simulink model "RobotDelta"  (R2025b)
settings: Solver=VariableStepAuto  StartTime=0.0  StopTime=10.0  RelTol=1e-3
model workspace: external: MATLAB File RobotDelta_DataFile.m (data not in the file)
undefined symbols (not defined in the file or in its folder): smiData, X, Y, Z
libraries: sm_lib x265, nesl_utility x1
(part 4 of 5)

== system RobotDelta/Mat_Bich_8mm_8_RIGID ==
  ReferenceFrame : sm_lib/Frames and Transforms/Reference Frame
  Solid : sm_lib/Body Elements/File Solid  ExtGeomFileName=Mat_Bich_8mm_Default_sldprt.STEP  UnitType=FromFile  ExtGeomFileUnits=m  StepReaderType=HEX  ExportConvexHullGeometry=off  InertiaType=Custom  BasedOnType=DensityFromFile  Density=1000  DensityUnits=kg/m^3  Mass=smiData.Solid(12).mass  MassUnits=kg  CenterOfMass=smiData.Solid(12).CoM  CenterOfMassUnits=mm  MomentsOfInertia=smiData.Solid(12).MoI  MomentsOfInertiaUnits=kg*mm^2  ProductsOfInertia=smiData.Solid(12).PoI  ProductsOfInertiaUnits=kg*mm^2  GraphicType=FromGeometry  MarkerShape=Sphere  MarkerSize=10  GraphicVisPropType=SimpleVisualProperties  GraphicDiffuseColor=smiData.Solid(12).color  GraphicOpacity=smiData.Solid(12).opacity  GraphicSpecularColor=[0.5 0.5 0.5 1.0]  GraphicAmbientColor=[0.15 0.15 0.15 1.0]  GraphicEmissiveColor=[0.0 0.0 0.0 1.0]  GraphicShininess=75  DoExposeReferenceFrame=on  SerializedFrames=<Frames/>
  Transform : sm_lib/Frames and Transforms/Rigid Transform  RotationMethod=ArbitraryAxis  FollAlignAxisA=+X  BaseAlignAxisA=+Y  FollAlignAxisB=+Y  BaseAlignAxisB=+Z  RotationStandardAxis=+Z  RotationAngle=smiData.RigidTransform(56).angle  RotationAngleUnits=rad  RotationArbitraryAxis=smiData.RigidTransform(56).axis  RotationSequenceAxes=FollowerAxes  RotationSequence=XYX  RotationSequenceAngles=[0 0 0]  RotationSequenceAnglesUnits=deg  RotationMatrix=[1 0 0;0 1 0;0 0 1]  Quaternion=[1 0 0 0]  TranslationMethod=Cartesian  TranslationCartesianOffset=smiData.RigidTransform(56).translation  TranslationCartesianOffsetUnits=mm  TranslationStandardAxis=+Z  TranslationStandardOffset=0  TranslationStandardOffsetUnits=m  TranslationROffset=0  TranslationROffsetUnits=m  TranslationThetaOffset=0  TranslationThetaOffsetUnits=deg  TranslationZOffset=0  TranslationZOffsetUnits=m
  Transform1 : sm_lib/Frames and Transforms/Rigid Transform  RotationMethod=ArbitraryAxis  FollAlignAxisA=+X  BaseAlignAxisA=+Y  FollAlignAxisB=+Y  BaseAlignAxisB=+Z  RotationStandardAxis=+Z  RotationAngle=smiData.RigidTransform(58).angle  RotationAngleUnits=rad  RotationArbitraryAxis=smiData.RigidTransform(58).axis  RotationSequenceAxes=FollowerAxes  RotationSequence=XYX  RotationSequenceAngles=[0 0 0]  RotationSequenceAnglesUnits=deg  RotationMatrix=[1 0 0;0 1 0;0 0 1]  Quaternion=[1 0 0 0]  TranslationMethod=Cartesian  TranslationCartesianOffset=smiData.RigidTransform(58).translation  TranslationCartesianOffsetUnits=mm  TranslationStandardAxis=+Z  TranslationStandardOffset=0  TranslationStandardOffsetUnits=m  TranslationROffset=0  TranslationROffsetUnits=m  TranslationThetaOffset=0  TranslationThetaOffsetUnits=deg  TranslationZOffset=0  TranslationZOffsetUnits=m
  F : PMIOPort  Side=Left
  F1 : PMIOPort  Port=2  Side=Left
  connections:
  Solid/RConn1 -- ReferenceFrame/RConn1 -- Transform/LConn1 -- Transform1/LConn1
  Transform/RConn1 -- F/RConn1
  Transform1/RConn1 -- F1/RConn1

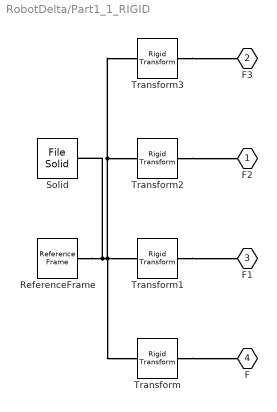
== system RobotDelta/Part1_1_RIGID ==
  ReferenceFrame : sm_lib/Frames and Transforms/Reference Frame
  Solid : sm_lib/Body Elements/File Solid  ExtGeomFileName=Part1_Default_sldprt.STEP  UnitType=FromFile  ExtGeomFileUnits=m  StepReaderType=HEX  ExportConvexHullGeometry=off  InertiaType=Custom  BasedOnType=DensityFromFile  Density=1000  DensityUnits=kg/m^3  Mass=smiData.Solid(10).mass  MassUnits=kg  CenterOfMass=smiData.Solid(10).CoM  CenterOfMassUnits=mm  MomentsOfInertia=smiData.Solid(10).MoI  MomentsOfInertiaUnits=kg*mm^2  ProductsOfInertia=smiData.Solid(10).PoI  ProductsOfInertiaUnits=kg*mm^2  GraphicType=FromGeometry  MarkerShape=Sphere  MarkerSize=10  GraphicVisPropType=SimpleVisualProperties  GraphicDiffuseColor=smiData.Solid(10).color  GraphicOpacity=smiData.Solid(10).opacity  GraphicSpecularColor=[0.5 0.5 0.5 1.0]  GraphicAmbientColor=[0.15 0.15 0.15 1.0]  GraphicEmissiveColor=[0.0 0.0 0.0 1.0]  GraphicShininess=75  DoExposeReferenceFrame=on  SerializedFrames=<Frames/>
  Transform : sm_lib/Frames and Transforms/Rigid Transform  RotationMethod=ArbitraryAxis  FollAlignAxisA=+X  BaseAlignAxisA=+Y  FollAlignAxisB=+Y  BaseAlignAxisB=+Z  RotationStandardAxis=+Z  RotationAngle=smiData.RigidTransform(43).angle  RotationAngleUnits=rad  RotationArbitraryAxis=smiData.RigidTransform(43).axis  RotationSequenceAxes=FollowerAxes  RotationSequence=XYX  RotationSequenceAngles=[0 0 0]  RotationSequenceAnglesUnits=deg  RotationMatrix=[1 0 0;0 1 0;0 0 1]  Quaternion=[1 0 0 0]  TranslationMethod=Cartesian  TranslationCartesianOffset=smiData.RigidTransform(43).translation  TranslationCartesianOffsetUnits=mm  TranslationStandardAxis=+Z  TranslationStandardOffset=0  TranslationStandardOffsetUnits=m  TranslationROffset=0  TranslationROffsetUnits=m  TranslationThetaOffset=0  TranslationThetaOffsetUnits=deg  TranslationZOffset=0  TranslationZOffsetUnits=m
  Transform1 : sm_lib/Frames and Transforms/Rigid Transform  RotationMethod=ArbitraryAxis  FollAlignAxisA=+X  BaseAlignAxisA=+Y  FollAlignAxisB=+Y  BaseAlignAxisB=+Z  RotationStandardAxis=+Z  RotationAngle=smiData.RigidTransform(49).angle  RotationAngleUnits=rad  RotationArbitraryAxis=smiData.RigidTransform(49).axis  RotationSequenceAxes=FollowerAxes  RotationSequence=XYX  RotationSequenceAngles=[0 0 0]  RotationSequenceAnglesUnits=deg  RotationMatrix=[1 0 0;0 1 0;0 0 1]  Quaternion=[1 0 0 0]  TranslationMethod=Cartesian  TranslationCartesianOffset=smiData.RigidTransform(49).translation  TranslationCartesianOffsetUnits=mm  TranslationStandardAxis=+Z  TranslationStandardOffset=0  TranslationStandardOffsetUnits=m  TranslationROffset=0  TranslationROffsetUnits=m  TranslationThetaOffset=0  TranslationThetaOffsetUnits=deg  TranslationZOffset=0  TranslationZOffsetUnits=m
  Transform2 : sm_lib/Frames and Transforms/Rigid Transform  RotationMethod=ArbitraryAxis  FollAlignAxisA=+X  BaseAlignAxisA=+Y  FollAlignAxisB=+Y  BaseAlignAxisB=+Z  RotationStandardAxis=+Z  RotationAngle=smiData.RigidTransform(91).angle  RotationAngleUnits=rad  RotationArbitraryAxis=smiData.RigidTransform(91).axis  RotationSequenceAxes=FollowerAxes  RotationSequence=XYX  RotationSequenceAngles=[0 0 0]  RotationSequenceAnglesUnits=deg  RotationMatrix=[1 0 0;0 1 0;0 0 1]  Quaternion=[1 0 0 0]  TranslationMethod=Cartesian  TranslationCartesianOffset=smiData.RigidTransform(91).translation  TranslationCartesianOffsetUnits=mm  TranslationStandardAxis=+Z  TranslationStandardOffset=0  TranslationStandardOffsetUnits=m  TranslationROffset=0  TranslationROffsetUnits=m  TranslationThetaOffset=0  TranslationThetaOffsetUnits=deg  TranslationZOffset=0  TranslationZOffsetUnits=m
  Transform3 : sm_lib/Frames and Transforms/Rigid Transform  RotationMethod=ArbitraryAxis  FollAlignAxisA=+X  BaseAlignAxisA=+Y  FollAlignAxisB=+Y  BaseAlignAxisB=+Z  RotationStandardAxis=+Z  RotationAngle=smiData.RigidTransform(94).angle  RotationAngleUnits=rad  RotationArbitraryAxis=smiData.RigidTransform(94).axis  RotationSequenceAxes=FollowerAxes  RotationSequence=XYX  RotationSequenceAngles=[0 0 0]  RotationSequenceAnglesUnits=deg  RotationMatrix=[1 0 0;0 1 0;0 0 1]  Quaternion=[1 0 0 0]  TranslationMethod=Cartesian  TranslationCartesianOffset=smiData.RigidTransform(94).translation  TranslationCartesianOffsetUnits=mm  TranslationStandardAxis=+Z  TranslationStandardOffset=0  TranslationStandardOffsetUnits=m  TranslationROffset=0  TranslationROffsetUnits=m  TranslationThetaOffset=0  TranslationThetaOffsetUnits=deg  TranslationZOffset=0  TranslationZOffsetUnits=m
  F2 : PMIOPort  Side=Left
  F3 : PMIOPort  Port=2  Side=Left
  F1 : PMIOPort  Port=3  Side=Left
  F : PMIOPort  Port=4  Side=Left
  connections:
  Solid/RConn1 -- ReferenceFrame/RConn1 -- Transform2/LConn1 -- Transform3/LConn1 -- Transform/LConn1 -- Transform1/LConn1
  Transform/RConn1 -- F/RConn1
  Transform1/RConn1 -- F1/RConn1
  Transform2/RConn1 -- F2/RConn1
  Transform3/RConn1 -- F3/RConn1

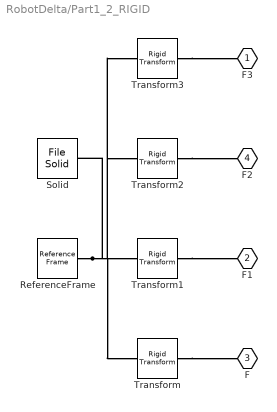
== system RobotDelta/Part1_2_RIGID ==
  ReferenceFrame : sm_lib/Frames and Transforms/Reference Frame
  Solid : sm_lib/Body Elements/File Solid  ExtGeomFileName=Part1_Default_sldprt.STEP  UnitType=FromFile  ExtGeomFileUnits=m  StepReaderType=HEX  ExportConvexHullGeometry=off  InertiaType=Custom  BasedOnType=DensityFromFile  Density=1000  DensityUnits=kg/m^3  Mass=smiData.Solid(10).mass  MassUnits=kg  CenterOfMass=smiData.Solid(10).CoM  CenterOfMassUnits=mm  MomentsOfInertia=smiData.Solid(10).MoI  MomentsOfInertiaUnits=kg*mm^2  ProductsOfInertia=smiData.Solid(10).PoI  ProductsOfInertiaUnits=kg*mm^2  GraphicType=FromGeometry  MarkerShape=Sphere  MarkerSize=10  GraphicVisPropType=SimpleVisualProperties  GraphicDiffuseColor=smiData.Solid(10).color  GraphicOpacity=smiData.Solid(10).opacity  GraphicSpecularColor=[0.5 0.5 0.5 1.0]  GraphicAmbientColor=[0.15 0.15 0.15 1.0]  GraphicEmissiveColor=[0.0 0.0 0.0 1.0]  GraphicShininess=75  DoExposeReferenceFrame=on  SerializedFrames=<Frames/>
  Transform : sm_lib/Frames and Transforms/Rigid Transform  RotationMethod=ArbitraryAxis  FollAlignAxisA=+X  BaseAlignAxisA=+Y  FollAlignAxisB=+Y  BaseAlignAxisB=+Z  RotationStandardAxis=+Z  RotationAngle=smiData.RigidTransform(51).angle  RotationAngleUnits=rad  RotationArbitraryAxis=smiData.RigidTransform(51).axis  RotationSequenceAxes=FollowerAxes  RotationSequence=XYX  RotationSequenceAngles=[0 0 0]  RotationSequenceAnglesUnits=deg  RotationMatrix=[1 0 0;0 1 0;0 0 1]  Quaternion=[1 0 0 0]  TranslationMethod=Cartesian  TranslationCartesianOffset=smiData.RigidTransform(51).translation  TranslationCartesianOffsetUnits=mm  TranslationStandardAxis=+Z  TranslationStandardOffset=0  TranslationStandardOffsetUnits=m  TranslationROffset=0  TranslationROffsetUnits=m  TranslationThetaOffset=0  TranslationThetaOffsetUnits=deg  TranslationZOffset=0  TranslationZOffsetUnits=m
  Transform1 : sm_lib/Frames and Transforms/Rigid Transform  RotationMethod=ArbitraryAxis  FollAlignAxisA=+X  BaseAlignAxisA=+Y  FollAlignAxisB=+Y  BaseAlignAxisB=+Z  RotationStandardAxis=+Z  RotationAngle=smiData.RigidTransform(55).angle  RotationAngleUnits=rad  RotationArbitraryAxis=smiData.RigidTransform(55).axis  RotationSequenceAxes=FollowerAxes  RotationSequence=XYX  RotationSequenceAngles=[0 0 0]  RotationSequenceAnglesUnits=deg  RotationMatrix=[1 0 0;0 1 0;0 0 1]  Quaternion=[1 0 0 0]  TranslationMethod=Cartesian  TranslationCartesianOffset=smiData.RigidTransform(55).translation  TranslationCartesianOffsetUnits=mm  TranslationStandardAxis=+Z  TranslationStandardOffset=0  TranslationStandardOffsetUnits=m  TranslationROffset=0  TranslationROffsetUnits=m  TranslationThetaOffset=0  TranslationThetaOffsetUnits=deg  TranslationZOffset=0  TranslationZOffsetUnits=m
  Transform2 : sm_lib/Frames and Transforms/Rigid Transform  RotationMethod=ArbitraryAxis  FollAlignAxisA=+X  BaseAlignAxisA=+Y  FollAlignAxisB=+Y  BaseAlignAxisB=+Z  RotationStandardAxis=+Z  RotationAngle=smiData.RigidTransform(95).angle  RotationAngleUnits=rad  RotationArbitraryAxis=smiData.RigidTransform(95).axis  RotationSequenceAxes=FollowerAxes  RotationSequence=XYX  RotationSequenceAngles=[0 0 0]  RotationSequenceAnglesUnits=deg  RotationMatrix=[1 0 0;0 1 0;0 0 1]  Quaternion=[1 0 0 0]  TranslationMethod=Cartesian  TranslationCartesianOffset=smiData.RigidTransform(95).translation  TranslationCartesianOffsetUnits=mm  TranslationStandardAxis=+Z  TranslationStandardOffset=0  TranslationStandardOffsetUnits=m  TranslationROffset=0  TranslationROffsetUnits=m  TranslationThetaOffset=0  TranslationThetaOffsetUnits=deg  TranslationZOffset=0  TranslationZOffsetUnits=m
  Transform3 : sm_lib/Frames and Transforms/Rigid Transform  RotationMethod=ArbitraryAxis  FollAlignAxisA=+X  BaseAlignAxisA=+Y  FollAlignAxisB=+Y  BaseAlignAxisB=+Z  RotationStandardAxis=+Z  RotationAngle=smiData.RigidTransform(98).angle  RotationAngleUnits=rad  RotationArbitraryAxis=smiData.RigidTransform(98).axis  RotationSequenceAxes=FollowerAxes  RotationSequence=XYX  RotationSequenceAngles=[0 0 0]  RotationSequenceAnglesUnits=deg  RotationMatrix=[1 0 0;0 1 0;0 0 1]  Quaternion=[1 0 0 0]  TranslationMethod=Cartesian  TranslationCartesianOffset=smiData.RigidTransform(98).translation  TranslationCartesianOffsetUnits=mm  TranslationStandardAxis=+Z  TranslationStandardOffset=0  TranslationStandardOffsetUnits=m  TranslationROffset=0  TranslationROffsetUnits=m  TranslationThetaOffset=0  TranslationThetaOffsetUnits=deg  TranslationZOffset=0  TranslationZOffsetUnits=m
  F3 : PMIOPort  Side=Left
  F1 : PMIOPort  Port=2  Side=Left
  F : PMIOPort  Port=3  Side=Left
  F2 : PMIOPort  Port=4  Side=Left
  connections:
  Solid/RConn1 -- ReferenceFrame/RConn1 -- Transform/LConn1 -- Transform1/LConn1 -- Transform2/LConn1 -- Transform3/LConn1
  Transform/RConn1 -- F/RConn1
  Transform1/RConn1 -- F1/RConn1
  Transform2/RConn1 -- F2/RConn1
  Transform3/RConn1 -- F3/RConn1

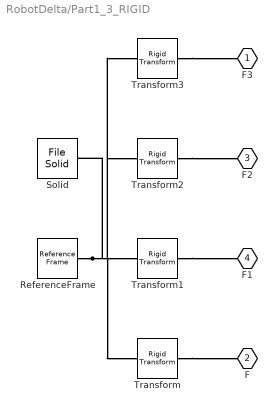
== system RobotDelta/Part1_3_RIGID ==
  ReferenceFrame : sm_lib/Frames and Transforms/Reference Frame
  Solid : sm_lib/Body Elements/File Solid  ExtGeomFileName=Part1_Default_sldprt.STEP  UnitType=FromFile  ExtGeomFileUnits=m  StepReaderType=HEX  ExportConvexHullGeometry=off  InertiaType=Custom  BasedOnType=DensityFromFile  Density=1000  DensityUnits=kg/m^3  Mass=smiData.Solid(10).mass  MassUnits=kg  CenterOfMass=smiData.Solid(10).CoM  CenterOfMassUnits=mm  MomentsOfInertia=smiData.Solid(10).MoI  MomentsOfInertiaUnits=kg*mm^2  ProductsOfInertia=smiData.Solid(10).PoI  ProductsOfInertiaUnits=kg*mm^2  GraphicType=FromGeometry  MarkerShape=Sphere  MarkerSize=10  GraphicVisPropType=SimpleVisualProperties  GraphicDiffuseColor=smiData.Solid(10).color  GraphicOpacity=smiData.Solid(10).opacity  GraphicSpecularColor=[0.5 0.5 0.5 1.0]  GraphicAmbientColor=[0.15 0.15 0.15 1.0]  GraphicEmissiveColor=[0.0 0.0 0.0 1.0]  GraphicShininess=75  DoExposeReferenceFrame=on  SerializedFrames=<Frames/>
  Transform : sm_lib/Frames and Transforms/Rigid Transform  RotationMethod=ArbitraryAxis  FollAlignAxisA=+X  BaseAlignAxisA=+Y  FollAlignAxisB=+Y  BaseAlignAxisB=+Z  RotationStandardAxis=+Z  RotationAngle=smiData.RigidTransform(33).angle  RotationAngleUnits=rad  RotationArbitraryAxis=smiData.RigidTransform(33).axis  RotationSequenceAxes=FollowerAxes  RotationSequence=XYX  RotationSequenceAngles=[0 0 0]  RotationSequenceAnglesUnits=deg  RotationMatrix=[1 0 0;0 1 0;0 0 1]  Quaternion=[1 0 0 0]  TranslationMethod=Cartesian  TranslationCartesianOffset=smiData.RigidTransform(33).translation  TranslationCartesianOffsetUnits=mm  TranslationStandardAxis=+Z  TranslationStandardOffset=0  TranslationStandardOffsetUnits=m  TranslationROffset=0  TranslationROffsetUnits=m  TranslationThetaOffset=0  TranslationThetaOffsetUnits=deg  TranslationZOffset=0  TranslationZOffsetUnits=m
  Transform1 : sm_lib/Frames and Transforms/Rigid Transform  RotationMethod=ArbitraryAxis  FollAlignAxisA=+X  BaseAlignAxisA=+Y  FollAlignAxisB=+Y  BaseAlignAxisB=+Z  RotationStandardAxis=+Z  RotationAngle=smiData.RigidTransform(37).angle  RotationAngleUnits=rad  RotationArbitraryAxis=smiData.RigidTransform(37).axis  RotationSequenceAxes=FollowerAxes  RotationSequence=XYX  RotationSequenceAngles=[0 0 0]  RotationSequenceAnglesUnits=deg  RotationMatrix=[1 0 0;0 1 0;0 0 1]  Quaternion=[1 0 0 0]  TranslationMethod=Cartesian  TranslationCartesianOffset=smiData.RigidTransform(37).translation  TranslationCartesianOffsetUnits=mm  TranslationStandardAxis=+Z  TranslationStandardOffset=0  TranslationStandardOffsetUnits=m  TranslationROffset=0  TranslationROffsetUnits=m  TranslationThetaOffset=0  TranslationThetaOffsetUnits=deg  TranslationZOffset=0  TranslationZOffsetUnits=m
  Transform2 : sm_lib/Frames and Transforms/Rigid Transform  RotationMethod=ArbitraryAxis  FollAlignAxisA=+X  BaseAlignAxisA=+Y  FollAlignAxisB=+Y  BaseAlignAxisB=+Z  RotationStandardAxis=+Z  RotationAngle=smiData.RigidTransform(99).angle  RotationAngleUnits=rad  RotationArbitraryAxis=smiData.RigidTransform(99).axis  RotationSequenceAxes=FollowerAxes  RotationSequence=XYX  RotationSequenceAngles=[0 0 0]  RotationSequenceAnglesUnits=deg  RotationMatrix=[1 0 0;0 1 0;0 0 1]  Quaternion=[1 0 0 0]  TranslationMethod=Cartesian  TranslationCartesianOffset=smiData.RigidTransform(99).translation  TranslationCartesianOffsetUnits=mm  TranslationStandardAxis=+Z  TranslationStandardOffset=0  TranslationStandardOffsetUnits=m  TranslationROffset=0  TranslationROffsetUnits=m  TranslationThetaOffset=0  TranslationThetaOffsetUnits=deg  TranslationZOffset=0  TranslationZOffsetUnits=m
  Transform3 : sm_lib/Frames and Transforms/Rigid Transform  RotationMethod=ArbitraryAxis  FollAlignAxisA=+X  BaseAlignAxisA=+Y  FollAlignAxisB=+Y  BaseAlignAxisB=+Z  RotationStandardAxis=+Z  RotationAngle=smiData.RigidTransform(102).angle  RotationAngleUnits=rad  RotationArbitraryAxis=smiData.RigidTransform(102).axis  RotationSequenceAxes=FollowerAxes  RotationSequence=XYX  RotationSequenceAngles=[0 0 0]  RotationSequenceAnglesUnits=deg  RotationMatrix=[1 0 0;0 1 0;0 0 1]  Quaternion=[1 0 0 0]  TranslationMethod=Cartesian  TranslationCartesianOffset=smiData.RigidTransform(102).translation  TranslationCartesianOffsetUnits=mm  TranslationStandardAxis=+Z  TranslationStandardOffset=0  TranslationStandardOffsetUnits=m  TranslationROffset=0  TranslationROffsetUnits=m  TranslationThetaOffset=0  TranslationThetaOffsetUnits=deg  TranslationZOffset=0  TranslationZOffsetUnits=m
  F3 : PMIOPort  Side=Left
  F : PMIOPort  Port=2  Side=Left
  F2 : PMIOPort  Port=3  Side=Left
  F1 : PMIOPort  Port=4  Side=Right
  connections:
  Solid/RConn1 -- ReferenceFrame/RConn1 -- Transform/LConn1 -- Transform1/LConn1 -- Transform2/LConn1 -- Transform3/LConn1
  Transform/RConn1 -- F/RConn1
  Transform1/RConn1 -- F1/RConn1
  Transform2/RConn1 -- F2/RConn1
  Transform3/RConn1 -- F3/RConn1

== system RobotDelta/ThanhTruyen_450mm_1_RIGID ==
  ReferenceFrame : sm_lib/Frames and Transforms/Reference Frame
  Solid : sm_lib/Body Elements/File Solid  ExtGeomFileName=ThanhTruyen_450mm_Default_sldprt.STEP  UnitType=FromFile  ExtGeomFileUnits=m  StepReaderType=HEX  ExportConvexHullGeometry=off  InertiaType=Custom  BasedOnType=DensityFromFile  Density=1000  DensityUnits=kg/m^3  Mass=smiData.Solid(3).mass  MassUnits=kg  CenterOfMass=smiData.Solid(3).CoM  CenterOfMassUnits=mm  MomentsOfInertia=smiData.Solid(3).MoI  MomentsOfInertiaUnits=kg*mm^2  ProductsOfInertia=smiData.Solid(3).PoI  ProductsOfInertiaUnits=kg*mm^2  GraphicType=FromGeometry  MarkerShape=Sphere  MarkerSize=10  GraphicVisPropType=SimpleVisualProperties  GraphicDiffuseColor=smiData.Solid(3).color  GraphicOpacity=smiData.Solid(3).opacity  GraphicSpecularColor=[0.5 0.5 0.5 1.0]  GraphicAmbientColor=[0.15 0.15 0.15 1.0]  GraphicEmissiveColor=[0.0 0.0 0.0 1.0]  GraphicShininess=75  DoExposeReferenceFrame=on  SerializedFrames=<Frames/>
  Transform : sm_lib/Frames and Transforms/Rigid Transform  RotationMethod=ArbitraryAxis  FollAlignAxisA=+X  BaseAlignAxisA=+Y  FollAlignAxisB=+Y  BaseAlignAxisB=+Z  RotationStandardAxis=+Z  RotationAngle=smiData.RigidTransform(64).angle  RotationAngleUnits=rad  RotationArbitraryAxis=smiData.RigidTransform(64).axis  RotationSequenceAxes=FollowerAxes  RotationSequence=XYX  RotationSequenceAngles=[0 0 0]  RotationSequenceAnglesUnits=deg  RotationMatrix=[1 0 0;0 1 0;0 0 1]  Quaternion=[1 0 0 0]  TranslationMethod=Cartesian  TranslationCartesianOffset=smiData.RigidTransform(64).translation  TranslationCartesianOffsetUnits=mm  TranslationStandardAxis=+Z  TranslationStandardOffset=0  TranslationStandardOffsetUnits=m  TranslationROffset=0  TranslationROffsetUnits=m  TranslationThetaOffset=0  TranslationThetaOffsetUnits=deg  TranslationZOffset=0  TranslationZOffsetUnits=m
  Transform1 : sm_lib/Frames and Transforms/Rigid Transform  RotationMethod=ArbitraryAxis  FollAlignAxisA=+X  BaseAlignAxisA=+Y  FollAlignAxisB=+Y  BaseAlignAxisB=+Z  RotationStandardAxis=+Z  RotationAngle=smiData.RigidTransform(80).angle  RotationAngleUnits=rad  RotationArbitraryAxis=smiData.RigidTransform(80).axis  RotationSequenceAxes=FollowerAxes  RotationSequence=XYX  RotationSequenceAngles=[0 0 0]  RotationSequenceAnglesUnits=deg  RotationMatrix=[1 0 0;0 1 0;0 0 1]  Quaternion=[1 0 0 0]  TranslationMethod=Cartesian  TranslationCartesianOffset=smiData.RigidTransform(80).translation  TranslationCartesianOffsetUnits=mm  TranslationStandardAxis=+Z  TranslationStandardOffset=0  TranslationStandardOffsetUnits=m  TranslationROffset=0  TranslationROffsetUnits=m  TranslationThetaOffset=0  TranslationThetaOffsetUnits=deg  TranslationZOffset=0  TranslationZOffsetUnits=m
  F1 : PMIOPort  Side=Left
  F : PMIOPort  Port=2  Side=Left
  connections:
  Solid/RConn1 -- ReferenceFrame/RConn1 -- Transform/LConn1 -- Transform1/LConn1
  Transform/RConn1 -- F/RConn1
  Transform1/RConn1 -- F1/RConn1

== system RobotDelta/ThanhTruyen_450mm_2_RIGID ==
  ReferenceFrame : sm_lib/Frames and Transforms/Reference Frame
  Solid : sm_lib/Body Elements/File Solid  ExtGeomFileName=ThanhTruyen_450mm_Default_sldprt.STEP  UnitType=FromFile  ExtGeomFileUnits=m  StepReaderType=HEX  ExportConvexHullGeometry=off  InertiaType=Custom  BasedOnType=DensityFromFile  Density=1000  DensityUnits=kg/m^3  Mass=smiData.Solid(3).mass  MassUnits=kg  CenterOfMass=smiData.Solid(3).CoM  CenterOfMassUnits=mm  MomentsOfInertia=smiData.Solid(3).MoI  MomentsOfInertiaUnits=kg*mm^2  ProductsOfInertia=smiData.Solid(3).PoI  ProductsOfInertiaUnits=kg*mm^2  GraphicType=FromGeometry  MarkerShape=Sphere  MarkerSize=10  GraphicVisPropType=SimpleVisualProperties  GraphicDiffuseColor=smiData.Solid(3).color  GraphicOpacity=smiData.Solid(3).opacity  GraphicSpecularColor=[0.5 0.5 0.5 1.0]  GraphicAmbientColor=[0.15 0.15 0.15 1.0]  GraphicEmissiveColor=[0.0 0.0 0.0 1.0]  GraphicShininess=75  DoExposeReferenceFrame=on  SerializedFrames=<Frames/>
  Transform : sm_lib/Frames and Transforms/Rigid Transform  RotationMethod=ArbitraryAxis  FollAlignAxisA=+X  BaseAlignAxisA=+Y  FollAlignAxisB=+Y  BaseAlignAxisB=+Z  RotationStandardAxis=+Z  RotationAngle=smiData.RigidTransform(60).angle  RotationAngleUnits=rad  RotationArbitraryAxis=smiData.RigidTransform(60).axis  RotationSequenceAxes=FollowerAxes  RotationSequence=XYX  RotationSequenceAngles=[0 0 0]  RotationSequenceAnglesUnits=deg  RotationMatrix=[1 0 0;0 1 0;0 0 1]  Quaternion=[1 0 0 0]  TranslationMethod=Cartesian  TranslationCartesianOffset=smiData.RigidTransform(60).translation  TranslationCartesianOffsetUnits=mm  TranslationStandardAxis=+Z  TranslationStandardOffset=0  TranslationStandardOffsetUnits=m  TranslationROffset=0  TranslationROffsetUnits=m  TranslationThetaOffset=0  TranslationThetaOffsetUnits=deg  TranslationZOffset=0  TranslationZOffsetUnits=m
  Transform1 : sm_lib/Frames and Transforms/Rigid Transform  RotationMethod=ArbitraryAxis  FollAlignAxisA=+X  BaseAlignAxisA=+Y  FollAlignAxisB=+Y  BaseAlignAxisB=+Z  RotationStandardAxis=+Z  RotationAngle=smiData.RigidTransform(84).angle  RotationAngleUnits=rad  RotationArbitraryAxis=smiData.RigidTransform(84).axis  RotationSequenceAxes=FollowerAxes  RotationSequence=XYX  RotationSequenceAngles=[0 0 0]  RotationSequenceAnglesUnits=deg  RotationMatrix=[1 0 0;0 1 0;0 0 1]  Quaternion=[1 0 0 0]  TranslationMethod=Cartesian  TranslationCartesianOffset=smiData.RigidTransform(84).translation  TranslationCartesianOffsetUnits=mm  TranslationStandardAxis=+Z  TranslationStandardOffset=0  TranslationStandardOffsetUnits=m  TranslationROffset=0  TranslationROffsetUnits=m  TranslationThetaOffset=0  TranslationThetaOffsetUnits=deg  TranslationZOffset=0  TranslationZOffsetUnits=m
  F1 : PMIOPort  Side=Left
  F : PMIOPort  Port=2  Side=Left
  connections:
  Solid/RConn1 -- ReferenceFrame/RConn1 -- Transform/LConn1 -- Transform1/LConn1
  Transform/RConn1 -- F/RConn1
  Transform1/RConn1 -- F1/RConn1

== system RobotDelta/ThanhTruyen_450mm_3_RIGID ==
  ReferenceFrame : sm_lib/Frames and Transforms/Reference Frame
  Solid : sm_lib/Body Elements/File Solid  ExtGeomFileName=ThanhTruyen_450mm_Default_sldprt.STEP  UnitType=FromFile  ExtGeomFileUnits=m  StepReaderType=HEX  ExportConvexHullGeometry=off  InertiaType=Custom  BasedOnType=DensityFromFile  Density=1000  DensityUnits=kg/m^3  Mass=smiData.Solid(3).mass  MassUnits=kg  CenterOfMass=smiData.Solid(3).CoM  CenterOfMassUnits=mm  MomentsOfInertia=smiData.Solid(3).MoI  MomentsOfInertiaUnits=kg*mm^2  ProductsOfInertia=smiData.Solid(3).PoI  ProductsOfInertiaUnits=kg*mm^2  GraphicType=FromGeometry  MarkerShape=Sphere  MarkerSize=10  GraphicVisPropType=SimpleVisualProperties  GraphicDiffuseColor=smiData.Solid(3).color  GraphicOpacity=smiData.Solid(3).opacity  GraphicSpecularColor=[0.5 0.5 0.5 1.0]  GraphicAmbientColor=[0.15 0.15 0.15 1.0]  GraphicEmissiveColor=[0.0 0.0 0.0 1.0]  GraphicShininess=75  DoExposeReferenceFrame=on  SerializedFrames=<Frames/>
  Transform : sm_lib/Frames and Transforms/Rigid Transform  RotationMethod=ArbitraryAxis  FollAlignAxisA=+X  BaseAlignAxisA=+Y  FollAlignAxisB=+Y  BaseAlignAxisB=+Z  RotationStandardAxis=+Z  RotationAngle=smiData.RigidTransform(2).angle  RotationAngleUnits=rad  RotationArbitraryAxis=smiData.RigidTransform(2).axis  RotationSequenceAxes=FollowerAxes  RotationSequence=XYX  RotationSequenceAngles=[0 0 0]  RotationSequenceAnglesUnits=deg  RotationMatrix=[1 0 0;0 1 0;0 0 1]  Quaternion=[1 0 0 0]  TranslationMethod=Cartesian  TranslationCartesianOffset=smiData.RigidTransform(2).translation  TranslationCartesianOffsetUnits=mm  TranslationStandardAxis=+Z  TranslationStandardOffset=0  TranslationStandardOffsetUnits=m  TranslationROffset=0  TranslationROffsetUnits=m  TranslationThetaOffset=0  TranslationThetaOffsetUnits=deg  TranslationZOffset=0  TranslationZOffsetUnits=m
  Transform1 : sm_lib/Frames and Transforms/Rigid Transform  RotationMethod=ArbitraryAxis  FollAlignAxisA=+X  BaseAlignAxisA=+Y  FollAlignAxisB=+Y  BaseAlignAxisB=+Z  RotationStandardAxis=+Z  RotationAngle=smiData.RigidTransform(76).angle  RotationAngleUnits=rad  RotationArbitraryAxis=smiData.RigidTransform(76).axis  RotationSequenceAxes=FollowerAxes  RotationSequence=XYX  RotationSequenceAngles=[0 0 0]  RotationSequenceAnglesUnits=deg  RotationMatrix=[1 0 0;0 1 0;0 0 1]  Quaternion=[1 0 0 0]  TranslationMethod=Cartesian  TranslationCartesianOffset=smiData.RigidTransform(76).translation  TranslationCartesianOffsetUnits=mm  TranslationStandardAxis=+Z  TranslationStandardOffset=0  TranslationStandardOffsetUnits=m  TranslationROffset=0  TranslationROffsetUnits=m  TranslationThetaOffset=0  TranslationThetaOffsetUnits=deg  TranslationZOffset=0  TranslationZOffsetUnits=m
  F : PMIOPort  Side=Left
  F1 : PMIOPort  Port=2  Side=Left
  connections:
  Solid/RConn1 -- ReferenceFrame/RConn1 -- Transform/LConn1 -- Transform1/LConn1
  Transform/RConn1 -- F/RConn1
  Transform1/RConn1 -- F1/RConn1

== system RobotDelta/ThanhTruyen_450mm_4_RIGID ==
  ReferenceFrame : sm_lib/Frames and Transforms/Reference Frame
  Solid : sm_lib/Body Elements/File Solid  ExtGeomFileName=ThanhTruyen_450mm_Default_sldprt.STEP  UnitType=FromFile  ExtGeomFileUnits=m  StepReaderType=HEX  ExportConvexHullGeometry=off  InertiaType=Custom  BasedOnType=DensityFromFile  Density=1000  DensityUnits=kg/m^3  Mass=smiData.Solid(3).mass  MassUnits=kg  CenterOfMass=smiData.Solid(3).CoM  CenterOfMassUnits=mm  MomentsOfInertia=smiData.Solid(3).MoI  MomentsOfInertiaUnits=kg*mm^2  ProductsOfInertia=smiData.Solid(3).PoI  ProductsOfInertiaUnits=kg*mm^2  GraphicType=FromGeometry  MarkerShape=Sphere  MarkerSize=10  GraphicVisPropType=SimpleVisualProperties  GraphicDiffuseColor=smiData.Solid(3).color  GraphicOpacity=smiData.Solid(3).opacity  GraphicSpecularColor=[0.5 0.5 0.5 1.0]  GraphicAmbientColor=[0.15 0.15 0.15 1.0]  GraphicEmissiveColor=[0.0 0.0 0.0 1.0]  GraphicShininess=75  DoExposeReferenceFrame=on  SerializedFrames=<Frames/>
  Transform : sm_lib/Frames and Transforms/Rigid Transform  RotationMethod=ArbitraryAxis  FollAlignAxisA=+X  BaseAlignAxisA=+Y  FollAlignAxisB=+Y  BaseAlignAxisB=+Z  RotationStandardAxis=+Z  RotationAngle=smiData.RigidTransform(4).angle  RotationAngleUnits=rad  RotationArbitraryAxis=smiData.RigidTransform(4).axis  RotationSequenceAxes=FollowerAxes  RotationSequence=XYX  RotationSequenceAngles=[0 0 0]  RotationSequenceAnglesUnits=deg  RotationMatrix=[1 0 0;0 1 0;0 0 1]  Quaternion=[1 0 0 0]  TranslationMethod=Cartesian  TranslationCartesianOffset=smiData.RigidTransform(4).translation  TranslationCartesianOffsetUnits=mm  TranslationStandardAxis=+Z  TranslationStandardOffset=0  TranslationStandardOffsetUnits=m  TranslationROffset=0  TranslationROffsetUnits=m  TranslationThetaOffset=0  TranslationThetaOffsetUnits=deg  TranslationZOffset=0  TranslationZOffsetUnits=m
  Transform1 : sm_lib/Frames and Transforms/Rigid Transform  RotationMethod=ArbitraryAxis  FollAlignAxisA=+X  BaseAlignAxisA=+Y  FollAlignAxisB=+Y  BaseAlignAxisB=+Z  RotationStandardAxis=+Z  RotationAngle=smiData.RigidTransform(72).angle  RotationAngleUnits=rad  RotationArbitraryAxis=smiData.RigidTransform(72).axis  RotationSequenceAxes=FollowerAxes  RotationSequence=XYX  RotationSequenceAngles=[0 0 0]  RotationSequenceAnglesUnits=deg  RotationMatrix=[1 0 0;0 1 0;0 0 1]  Quaternion=[1 0 0 0]  TranslationMethod=Cartesian  TranslationCartesianOffset=smiData.RigidTransform(72).translation  TranslationCartesianOffsetUnits=mm  TranslationStandardAxis=+Z  TranslationStandardOffset=0  TranslationStandardOffsetUnits=m  TranslationROffset=0  TranslationROffsetUnits=m  TranslationThetaOffset=0  TranslationThetaOffsetUnits=deg  TranslationZOffset=0  TranslationZOffsetUnits=m
  F : PMIOPort  Side=Left
  F1 : PMIOPort  Port=2  Side=Left
  connections:
  Solid/RConn1 -- ReferenceFrame/RConn1 -- Transform/LConn1 -- Transform1/LConn1
  Transform/RConn1 -- F/RConn1
  Transform1/RConn1 -- F1/RConn1

== system RobotDelta/ThanhTruyen_450mm_5_RIGID ==
  ReferenceFrame : sm_lib/Frames and Transforms/Reference Frame
  Solid : sm_lib/Body Elements/File Solid  ExtGeomFileName=ThanhTruyen_450mm_Default_sldprt.STEP  UnitType=FromFile  ExtGeomFileUnits=m  StepReaderType=HEX  ExportConvexHullGeometry=off  InertiaType=Custom  BasedOnType=DensityFromFile  Density=1000  DensityUnits=kg/m^3  Mass=smiData.Solid(3).mass  MassUnits=kg  CenterOfMass=smiData.Solid(3).CoM  CenterOfMassUnits=mm  MomentsOfInertia=smiData.Solid(3).MoI  MomentsOfInertiaUnits=kg*mm^2  ProductsOfInertia=smiData.Solid(3).PoI  ProductsOfInertiaUnits=kg*mm^2  GraphicType=FromGeometry  MarkerShape=Sphere  MarkerSize=10  GraphicVisPropType=SimpleVisualProperties  GraphicDiffuseColor=smiData.Solid(3).color  GraphicOpacity=smiData.Solid(3).opacity  GraphicSpecularColor=[0.5 0.5 0.5 1.0]  GraphicAmbientColor=[0.15 0.15 0.15 1.0]  GraphicEmissiveColor=[0.0 0.0 0.0 1.0]  GraphicShininess=75  DoExposeReferenceFrame=on  SerializedFrames=<Frames/>
  Transform : sm_lib/Frames and Transforms/Rigid Transform  RotationMethod=ArbitraryAxis  FollAlignAxisA=+X  BaseAlignAxisA=+Y  FollAlignAxisB=+Y  BaseAlignAxisB=+Z  RotationStandardAxis=+Z  RotationAngle=smiData.RigidTransform(6).angle  RotationAngleUnits=rad  RotationArbitraryAxis=smiData.RigidTransform(6).axis  RotationSequenceAxes=FollowerAxes  RotationSequence=XYX  RotationSequenceAngles=[0 0 0]  RotationSequenceAnglesUnits=deg  RotationMatrix=[1 0 0;0 1 0;0 0 1]  Quaternion=[1 0 0 0]  TranslationMethod=Cartesian  TranslationCartesianOffset=smiData.RigidTransform(6).translation  TranslationCartesianOffsetUnits=mm  TranslationStandardAxis=+Z  TranslationStandardOffset=0  TranslationStandardOffsetUnits=m  TranslationROffset=0  TranslationROffsetUnits=m  TranslationThetaOffset=0  TranslationThetaOffsetUnits=deg  TranslationZOffset=0  TranslationZOffsetUnits=m
  Transform1 : sm_lib/Frames and Transforms/Rigid Transform  RotationMethod=ArbitraryAxis  FollAlignAxisA=+X  BaseAlignAxisA=+Y  FollAlignAxisB=+Y  BaseAlignAxisB=+Z  RotationStandardAxis=+Z  RotationAngle=smiData.RigidTransform(68).angle  RotationAngleUnits=rad  RotationArbitraryAxis=smiData.RigidTransform(68).axis  RotationSequenceAxes=FollowerAxes  RotationSequence=XYX  RotationSequenceAngles=[0 0 0]  RotationSequenceAnglesUnits=deg  RotationMatrix=[1 0 0;0 1 0;0 0 1]  Quaternion=[1 0 0 0]  TranslationMethod=Cartesian  TranslationCartesianOffset=smiData.RigidTransform(68).translation  TranslationCartesianOffsetUnits=mm  TranslationStandardAxis=+Z  TranslationStandardOffset=0  TranslationStandardOffsetUnits=m  TranslationROffset=0  TranslationROffsetUnits=m  TranslationThetaOffset=0  TranslationThetaOffsetUnits=deg  TranslationZOffset=0  TranslationZOffsetUnits=m
  F1 : PMIOPort  Side=Left
  F : PMIOPort  Port=2  Side=Left
  connections:
  Solid/RConn1 -- ReferenceFrame/RConn1 -- Transform/LConn1 -- Transform1/LConn1
  Transform/RConn1 -- F/RConn1
  Transform1/RConn1 -- F1/RConn1

== system RobotDelta/ThanhTruyen_450mm_6_RIGID ==
  ReferenceFrame : sm_lib/Frames and Transforms/Reference Frame
  Solid : sm_lib/Body Elements/File Solid  ExtGeomFileName=ThanhTruyen_450mm_Default_sldprt.STEP  UnitType=FromFile  ExtGeomFileUnits=m  StepReaderType=HEX  ExportConvexHullGeometry=off  InertiaType=Custom  BasedOnType=DensityFromFile  Density=1000  DensityUnits=kg/m^3  Mass=smiData.Solid(3).mass  MassUnits=kg  CenterOfMass=smiData.Solid(3).CoM  CenterOfMassUnits=mm  MomentsOfInertia=smiData.Solid(3).MoI  MomentsOfInertiaUnits=kg*mm^2  ProductsOfInertia=smiData.Solid(3).PoI  ProductsOfInertiaUnits=kg*mm^2  GraphicType=FromGeometry  MarkerShape=Sphere  MarkerSize=10  GraphicVisPropType=SimpleVisualProperties  GraphicDiffuseColor=smiData.Solid(3).color  GraphicOpacity=smiData.Solid(3).opacity  GraphicSpecularColor=[0.5 0.5 0.5 1.0]  GraphicAmbientColor=[0.15 0.15 0.15 1.0]  GraphicEmissiveColor=[0.0 0.0 0.0 1.0]  GraphicShininess=75  DoExposeReferenceFrame=on  SerializedFrames=<Frames/>
  Transform : sm_lib/Frames and Transforms/Rigid Transform  RotationMethod=ArbitraryAxis  FollAlignAxisA=+X  BaseAlignAxisA=+Y  FollAlignAxisB=+Y  BaseAlignAxisB=+Z  RotationStandardAxis=+Z  RotationAngle=smiData.RigidTransform(8).angle  RotationAngleUnits=rad  RotationArbitraryAxis=smiData.RigidTransform(8).axis  RotationSequenceAxes=FollowerAxes  RotationSequence=XYX  RotationSequenceAngles=[0 0 0]  RotationSequenceAnglesUnits=deg  RotationMatrix=[1 0 0;0 1 0;0 0 1]  Quaternion=[1 0 0 0]  TranslationMethod=Cartesian  TranslationCartesianOffset=smiData.RigidTransform(8).translation  TranslationCartesianOffsetUnits=mm  TranslationStandardAxis=+Z  TranslationStandardOffset=0  TranslationStandardOffsetUnits=m  TranslationROffset=0  TranslationROffsetUnits=m  TranslationThetaOffset=0  TranslationThetaOffsetUnits=deg  TranslationZOffset=0  TranslationZOffsetUnits=m
  Transform1 : sm_lib/Frames and Transforms/Rigid Transform  RotationMethod=ArbitraryAxis  FollAlignAxisA=+X  BaseAlignAxisA=+Y  FollAlignAxisB=+Y  BaseAlignAxisB=+Z  RotationStandardAxis=+Z  RotationAngle=smiData.RigidTransform(88).angle  RotationAngleUnits=rad  RotationArbitraryAxis=smiData.RigidTransform(88).axis  RotationSequenceAxes=FollowerAxes  RotationSequence=XYX  RotationSequenceAngles=[0 0 0]  RotationSequenceAnglesUnits=deg  RotationMatrix=[1 0 0;0 1 0;0 0 1]  Quaternion=[1 0 0 0]  TranslationMethod=Cartesian  TranslationCartesianOffset=smiData.RigidTransform(88).translation  TranslationCartesianOffsetUnits=mm  TranslationStandardAxis=+Z  TranslationStandardOffset=0  TranslationStandardOffsetUnits=m  TranslationROffset=0  TranslationROffsetUnits=m  TranslationThetaOffset=0  TranslationThetaOffsetUnits=deg  TranslationZOffset=0  TranslationZOffsetUnits=m
  F1 : PMIOPort  Side=Left
  F : PMIOPort  Port=2  Side=Left
  connections:
  Solid/RConn1 -- ReferenceFrame/RConn1 -- Transform/LConn1 -- Transform1/LConn1
  Transform/RConn1 -- F/RConn1
  Transform1/RConn1 -- F1/RConn1

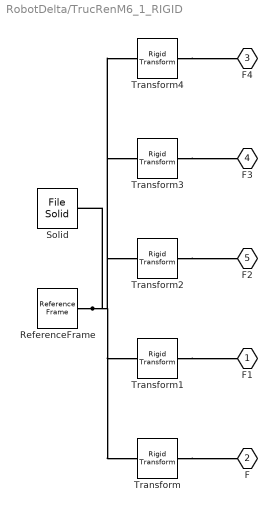
== system RobotDelta/TrucRenM6_1_RIGID ==
  ReferenceFrame : sm_lib/Frames and Transforms/Reference Frame
  Solid : sm_lib/Body Elements/File Solid  ExtGeomFileName=TrucRenM6_Default_sldprt.STEP  UnitType=FromFile  ExtGeomFileUnits=m  StepReaderType=HEX  ExportConvexHullGeometry=off  InertiaType=Custom  BasedOnType=DensityFromFile  Density=1000  DensityUnits=kg/m^3  Mass=smiData.Solid(5).mass  MassUnits=kg  CenterOfMass=smiData.Solid(5).CoM  CenterOfMassUnits=mm  MomentsOfInertia=smiData.Solid(5).MoI  MomentsOfInertiaUnits=kg*mm^2  ProductsOfInertia=smiData.Solid(5).PoI  ProductsOfInertiaUnits=kg*mm^2  GraphicType=FromGeometry  MarkerShape=Sphere  MarkerSize=10  GraphicVisPropType=SimpleVisualProperties  GraphicDiffuseColor=smiData.Solid(5).color  GraphicOpacity=smiData.Solid(5).opacity  GraphicSpecularColor=[0.5 0.5 0.5 1.0]  GraphicAmbientColor=[0.15 0.15 0.15 1.0]  GraphicEmissiveColor=[0.0 0.0 0.0 1.0]  GraphicShininess=75  DoExposeReferenceFrame=on  SerializedFrames=<Frames/>
  Transform : sm_lib/Frames and Transforms/Rigid Transform  RotationMethod=ArbitraryAxis  FollAlignAxisA=+X  BaseAlignAxisA=+Y  FollAlignAxisB=+Y  BaseAlignAxisB=+Z  RotationStandardAxis=+Z  RotationAngle=smiData.RigidTransform(36).angle  RotationAngleUnits=rad  RotationArbitraryAxis=smiData.RigidTransform(36).axis  RotationSequenceAxes=FollowerAxes  RotationSequence=XYX  RotationSequenceAngles=[0 0 0]  RotationSequenceAnglesUnits=deg  RotationMatrix=[1 0 0;0 1 0;0 0 1]  Quaternion=[1 0 0 0]  TranslationMethod=Cartesian  TranslationCartesianOffset=smiData.RigidTransform(36).translation  TranslationCartesianOffsetUnits=mm  TranslationStandardAxis=+Z  TranslationStandardOffset=0  TranslationStandardOffsetUnits=m  TranslationROffset=0  TranslationROffsetUnits=m  TranslationThetaOffset=0  TranslationThetaOffsetUnits=deg  TranslationZOffset=0  TranslationZOffsetUnits=m
  Transform1 : sm_lib/Frames and Transforms/Rigid Transform  RotationMethod=ArbitraryAxis  FollAlignAxisA=+X  BaseAlignAxisA=+Y  FollAlignAxisB=+Y  BaseAlignAxisB=+Z  RotationStandardAxis=+Z  RotationAngle=smiData.RigidTransform(40).angle  RotationAngleUnits=rad  RotationArbitraryAxis=smiData.RigidTransform(40).axis  RotationSequenceAxes=FollowerAxes  RotationSequence=XYX  RotationSequenceAngles=[0 0 0]  RotationSequenceAnglesUnits=deg  RotationMatrix=[1 0 0;0 1 0;0 0 1]  Quaternion=[1 0 0 0]  TranslationMethod=Cartesian  TranslationCartesianOffset=smiData.RigidTransform(40).translation  TranslationCartesianOffsetUnits=mm  TranslationStandardAxis=+Z  TranslationStandardOffset=0  TranslationStandardOffsetUnits=m  TranslationROffset=0  TranslationROffsetUnits=m  TranslationThetaOffset=0  TranslationThetaOffsetUnits=deg  TranslationZOffset=0  TranslationZOffsetUnits=m
  Transform2 : sm_lib/Frames and Transforms/Rigid Transform  RotationMethod=ArbitraryAxis  FollAlignAxisA=+X  BaseAlignAxisA=+Y  FollAlignAxisB=+Y  BaseAlignAxisB=+Z  RotationStandardAxis=+Z  RotationAngle=smiData.RigidTransform(103).angle  RotationAngleUnits=rad  RotationArbitraryAxis=smiData.RigidTransform(103).axis  RotationSequenceAxes=FollowerAxes  RotationSequence=XYX  RotationSequenceAngles=[0 0 0]  RotationSequenceAnglesUnits=deg  RotationMatrix=[1 0 0;0 1 0;0 0 1]  Quaternion=[1 0 0 0]  TranslationMethod=Cartesian  TranslationCartesianOffset=smiData.RigidTransform(103).translation  TranslationCartesianOffsetUnits=mm  TranslationStandardAxis=+Z  TranslationStandardOffset=0  TranslationStandardOffsetUnits=m  TranslationROffset=0  TranslationROffsetUnits=m  TranslationThetaOffset=0  TranslationThetaOffsetUnits=deg  TranslationZOffset=0  TranslationZOffsetUnits=m
  Transform3 : sm_lib/Frames and Transforms/Rigid Transform  RotationMethod=ArbitraryAxis  FollAlignAxisA=+X  BaseAlignAxisA=+Y  FollAlignAxisB=+Y  BaseAlignAxisB=+Z  RotationStandardAxis=+Z  RotationAngle=smiData.RigidTransform(105).angle  RotationAngleUnits=rad  RotationArbitraryAxis=smiData.RigidTransform(105).axis  RotationSequenceAxes=FollowerAxes  RotationSequence=XYX  RotationSequenceAngles=[0 0 0]  RotationSequenceAnglesUnits=deg  RotationMatrix=[1 0 0;0 1 0;0 0 1]  Quaternion=[1 0 0 0]  TranslationMethod=Cartesian  TranslationCartesianOffset=smiData.RigidTransform(105).translation  TranslationCartesianOffsetUnits=mm  TranslationStandardAxis=+Z  TranslationStandardOffset=0  TranslationStandardOffsetUnits=m  TranslationROffset=0  TranslationROffsetUnits=m  TranslationThetaOffset=0  TranslationThetaOffsetUnits=deg  TranslationZOffset=0  TranslationZOffsetUnits=m
  Transform4 : sm_lib/Frames and Transforms/Rigid Transform  RotationMethod=ArbitraryAxis  FollAlignAxisA=+X  BaseAlignAxisA=+Y  FollAlignAxisB=+Y  BaseAlignAxisB=+Z  RotationStandardAxis=+Z  RotationAngle=smiData.RigidTransform(107).angle  RotationAngleUnits=rad  RotationArbitraryAxis=smiData.RigidTransform(107).axis  RotationSequenceAxes=FollowerAxes  RotationSequence=XYX  RotationSequenceAngles=[0 0 0]  RotationSequenceAnglesUnits=deg  RotationMatrix=[1 0 0;0 1 0;0 0 1]  Quaternion=[1 0 0 0]  TranslationMethod=Cartesian  TranslationCartesianOffset=smiData.RigidTransform(107).translation  TranslationCartesianOffsetUnits=mm  TranslationStandardAxis=+Z  TranslationStandardOffset=0  TranslationStandardOffsetUnits=m  TranslationROffset=0  TranslationROffsetUnits=m  TranslationThetaOffset=0  TranslationThetaOffsetUnits=deg  TranslationZOffset=0  TranslationZOffsetUnits=m
  F1 : PMIOPort  Side=Left
  F : PMIOPort  Port=2  Side=Left
  F4 : PMIOPort  Port=3  Side=Right
  F3 : PMIOPort  Port=4  Side=Right
  F2 : PMIOPort  Port=5  Side=Right
  connections:
  Solid/RConn1 -- ReferenceFrame/RConn1 -- Transform/LConn1 -- Transform1/LConn1 -- Transform2/LConn1 -- Transform3/LConn1 -- Transform4/LConn1
  Transform/RConn1 -- F/RConn1
  Transform1/RConn1 -- F1/RConn1
  Transform2/RConn1 -- F2/RConn1
  Transform3/RConn1 -- F3/RConn1
  Transform4/RConn1 -- F4/RConn1

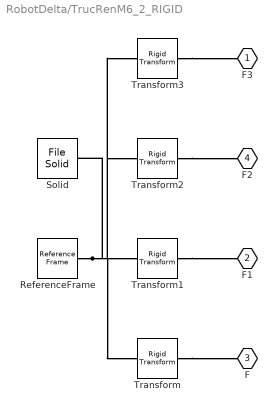
== system RobotDelta/TrucRenM6_2_RIGID ==
  ReferenceFrame : sm_lib/Frames and Transforms/Reference Frame
  Solid : sm_lib/Body Elements/File Solid  ExtGeomFileName=TrucRenM6_Default_sldprt.STEP  UnitType=FromFile  ExtGeomFileUnits=m  StepReaderType=HEX  ExportConvexHullGeometry=off  InertiaType=Custom  BasedOnType=DensityFromFile  Density=1000  DensityUnits=kg/m^3  Mass=smiData.Solid(5).mass  MassUnits=kg  CenterOfMass=smiData.Solid(5).CoM  CenterOfMassUnits=mm  MomentsOfInertia=smiData.Solid(5).MoI  MomentsOfInertiaUnits=kg*mm^2  ProductsOfInertia=smiData.Solid(5).PoI  ProductsOfInertiaUnits=kg*mm^2  GraphicType=FromGeometry  MarkerShape=Sphere  MarkerSize=10  GraphicVisPropType=SimpleVisualProperties  GraphicDiffuseColor=smiData.Solid(5).color  GraphicOpacity=smiData.Solid(5).opacity  GraphicSpecularColor=[0.5 0.5 0.5 1.0]  GraphicAmbientColor=[0.15 0.15 0.15 1.0]  GraphicEmissiveColor=[0.0 0.0 0.0 1.0]  GraphicShininess=75  DoExposeReferenceFrame=on  SerializedFrames=<Frames/>
  Transform : sm_lib/Frames and Transforms/Rigid Transform  RotationMethod=ArbitraryAxis  FollAlignAxisA=+X  BaseAlignAxisA=+Y  FollAlignAxisB=+Y  BaseAlignAxisB=+Z  RotationStandardAxis=+Z  RotationAngle=smiData.RigidTransform(53).angle  RotationAngleUnits=rad  RotationArbitraryAxis=smiData.RigidTransform(53).axis  RotationSequenceAxes=FollowerAxes  RotationSequence=XYX  RotationSequenceAngles=[0 0 0]  RotationSequenceAnglesUnits=deg  RotationMatrix=[1 0 0;0 1 0;0 0 1]  Quaternion=[1 0 0 0]  TranslationMethod=Cartesian  TranslationCartesianOffset=smiData.RigidTransform(53).translation  TranslationCartesianOffsetUnits=mm  TranslationStandardAxis=+Z  TranslationStandardOffset=0  TranslationStandardOffsetUnits=m  TranslationROffset=0  TranslationROffsetUnits=m  TranslationThetaOffset=0  TranslationThetaOffsetUnits=deg  TranslationZOffset=0  TranslationZOffsetUnits=m
  Transform1 : sm_lib/Frames and Transforms/Rigid Transform  RotationMethod=ArbitraryAxis  FollAlignAxisA=+X  BaseAlignAxisA=+Y  FollAlignAxisB=+Y  BaseAlignAxisB=+Z  RotationStandardAxis=+Z  RotationAngle=smiData.RigidTransform(57).angle  RotationAngleUnits=rad  RotationArbitraryAxis=smiData.RigidTransform(57).axis  RotationSequenceAxes=FollowerAxes  RotationSequence=XYX  RotationSequenceAngles=[0 0 0]  RotationSequenceAnglesUnits=deg  RotationMatrix=[1 0 0;0 1 0;0 0 1]  Quaternion=[1 0 0 0]  TranslationMethod=Cartesian  TranslationCartesianOffset=smiData.RigidTransform(57).translation  TranslationCartesianOffsetUnits=mm  TranslationStandardAxis=+Z  TranslationStandardOffset=0  TranslationStandardOffsetUnits=m  TranslationROffset=0  TranslationROffsetUnits=m  TranslationThetaOffset=0  TranslationThetaOffsetUnits=deg  TranslationZOffset=0  TranslationZOffsetUnits=m
  Transform2 : sm_lib/Frames and Transforms/Rigid Transform  RotationMethod=ArbitraryAxis  FollAlignAxisA=+X  BaseAlignAxisA=+Y  FollAlignAxisB=+Y  BaseAlignAxisB=+Z  RotationStandardAxis=+Z  RotationAngle=smiData.RigidTransform(109).angle  RotationAngleUnits=rad  RotationArbitraryAxis=smiData.RigidTransform(109).axis  RotationSequenceAxes=FollowerAxes  RotationSequence=XYX  RotationSequenceAngles=[0 0 0]  RotationSequenceAnglesUnits=deg  RotationMatrix=[1 0 0;0 1 0;0 0 1]  Quaternion=[1 0 0 0]  TranslationMethod=Cartesian  TranslationCartesianOffset=smiData.RigidTransform(109).translation  TranslationCartesianOffsetUnits=mm  TranslationStandardAxis=+Z  TranslationStandardOffset=0  TranslationStandardOffsetUnits=m  TranslationROffset=0  TranslationROffsetUnits=m  TranslationThetaOffset=0  TranslationThetaOffsetUnits=deg  TranslationZOffset=0  TranslationZOffsetUnits=m
  Transform3 : sm_lib/Frames and Transforms/Rigid Transform  RotationMethod=ArbitraryAxis  FollAlignAxisA=+X  BaseAlignAxisA=+Y  FollAlignAxisB=+Y  BaseAlignAxisB=+Z  RotationStandardAxis=+Z  RotationAngle=smiData.RigidTransform(111).angle  RotationAngleUnits=rad  RotationArbitraryAxis=smiData.RigidTransform(111).axis  RotationSequenceAxes=FollowerAxes  RotationSequence=XYX  RotationSequenceAngles=[0 0 0]  RotationSequenceAnglesUnits=deg  RotationMatrix=[1 0 0;0 1 0;0 0 1]  Quaternion=[1 0 0 0]  TranslationMethod=Cartesian  TranslationCartesianOffset=smiData.RigidTransform(111).translation  TranslationCartesianOffsetUnits=mm  TranslationStandardAxis=+Z  TranslationStandardOffset=0  TranslationStandardOffsetUnits=m  TranslationROffset=0  TranslationROffsetUnits=m  TranslationThetaOffset=0  TranslationThetaOffsetUnits=deg  TranslationZOffset=0  TranslationZOffsetUnits=m
  F3 : PMIOPort  Side=Right
  F1 : PMIOPort  Port=2  Side=Right
  F : PMIOPort  Port=3  Side=Right
  F2 : PMIOPort  Port=4  Side=Right
  connections:
  Solid/RConn1 -- ReferenceFrame/RConn1 -- Transform/LConn1 -- Transform1/LConn1 -- Transform2/LConn1 -- Transform3/LConn1
  Transform/RConn1 -- F/RConn1
  Transform1/RConn1 -- F1/RConn1
  Transform2/RConn1 -- F2/RConn1
  Transform3/RConn1 -- F3/RConn1
